simulink model "lab3"  (R2025b)
settings: Solver=FixedStepAuto  StartTime=0.0  StopTime=10.0  FixedStep=0.001  RelTol=1e-3
undefined symbols (not defined in the file): A, B, K, k, r
settings Model: Creator=Nickolay  LastModifiedBy=Nickolay

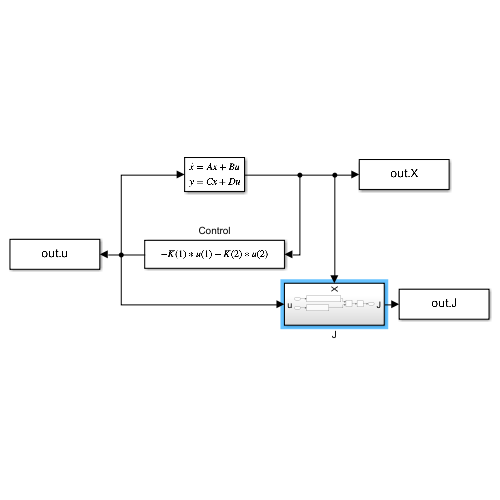
[thumbnail: Simulink's stored preview of the top-level diagram]
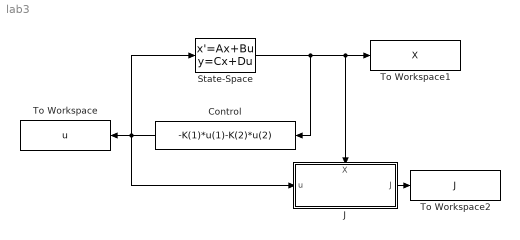
== system lab3 ==
  Control : Fcn  Expr=-K(1)*u(1)-K(2)*u(2)
  J : Subsystem
      settings: PortSchema="{\"entries\":[{\"content\":{\"sides\":[{\"content\":{\"connectorIds\":[\"In1\"]},\"type\":\"ConnectorPlacement.EquallySpacedRectSide\",\"uuid\":\"042fbab3-3dd3-4377-a165-f6b6937dec10\"},{\"content\":{\"connectorIds\":[\"Out1\"],\"side\":\"RIGHT\"},\"type\":\"ConnectorPlacement.EquallySpacedRectSide\",\"uuid\":\"7b0bef8b-880e-4cf3-8709-a0510a4e0f1d\"},{\"content\":{\"connectorIds\":[\"In2\"],\"side\":\"TOP\"},\"type\":\"ConnectorPlacement.EquallySpacedRectSide\",\"uuid\":\"acbcb399-af56-4bc0-9ffd-2cbaf38c24e1\"}]},\"type\":\"ConnectorPlacement.EquallySpacedConnector\",\"uuid\":\"690ac16e-4901-420e-baa7-8378651d93c9\"}],\"packageUris\":[\"http://schema.mathworks.com/mf0/Connector/R2020b\"],\"version\":\"1.0\"}"
  State-Space : StateSpace  A=A  B=B  C=eye(2)  D=[0; 0]  InitialCondition=[1; 0]
  To Workspace : ToWorkspace  VariableName=u  SaveFormat=Timeseries  SampleTime=-1
  To Workspace1 : ToWorkspace  VariableName=X  SaveFormat=Timeseries  SampleTime=-1
  To Workspace2 : ToWorkspace  VariableName=J  SaveFormat=Timeseries  SampleTime=-1
  wires:
  Control/1 -> J/1(u), To Workspace/1, State-Space/1
  State-Space/1 -> J/2(X), To Workspace1/1, Control/1
  J/1(J) -> To Workspace2/1

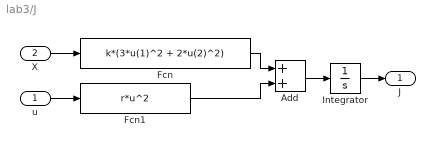
== system lab3/J ==
  u : Inport
  X : Inport  Port=2
  Add : Sum
  Fcn : Fcn  Expr=k*(3*u(1)^2 + 2*u(2)^2)
  Fcn1 : Fcn  Expr=r*u^2
  Integrator : Integrator
  J : Outport
  wires:
  Integrator/1 -> J/1
  X/1 -> Fcn/1
  u/1 -> Fcn1/1
  Fcn/1 -> Add/1
  Fcn1/1 -> Add/2
  Add/1 -> Integrator/1
